simulink model "simulation_ref"  (R2026a)
settings: Solver=ode45  StopTime=stop_time  MaxStep=0.05
values from neighbouring files (symbols this model uses):
  throttle_trim = T_trim/T_max    [main.m]
undefined symbols (not defined in the file or in its folder): gravity_earth
settings Model: Creator=darpansingh  LastModifiedBy=lilos

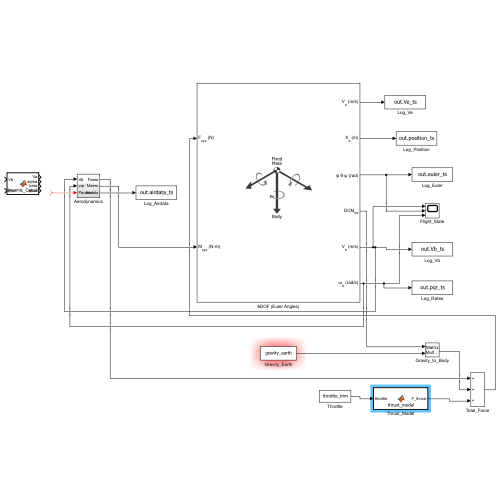
[thumbnail: Simulink's stored preview of the top-level diagram]
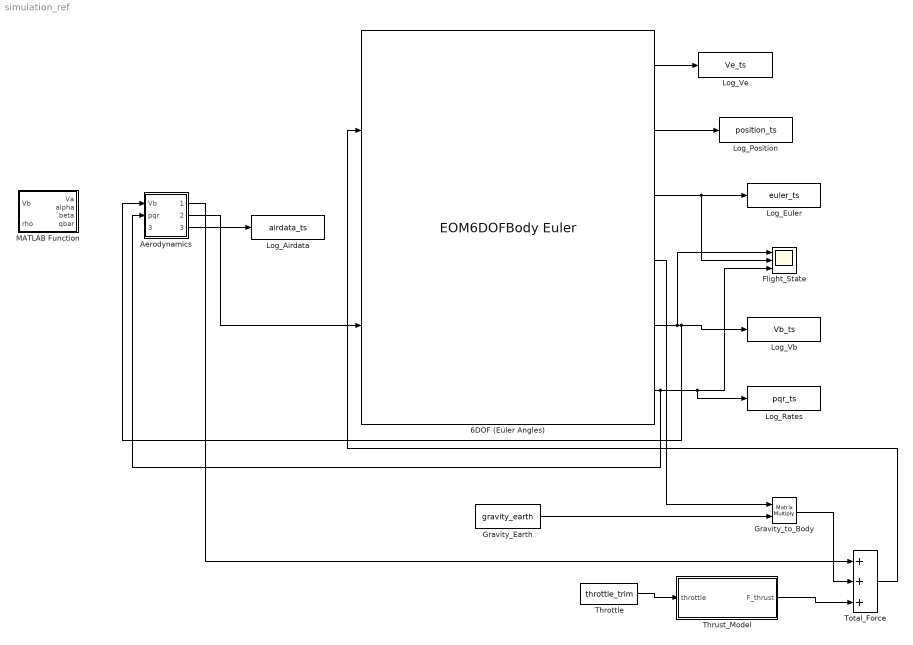
== system simulation_ref ==
  6DOF (Euler Angles) : EOM6DOFBodyEuler  xme_0=pos0  Vm_0=vel0  eul_0=euler0  pm_0=omega0  mass_0=mass  inertia=inertia
  Aerodynamics : Subsystem
  Flight_State : Scope  NumInputPorts=3
      settings: ActiveDisplayYMinimum=-1  ActiveDisplayYMaximum=1
  Gravity_Earth : Constant  Value=gravity_earth
  Gravity_to_Body : Product  Inputs=**  Multiplication=Matrix(*)
  Log_Airdata : ToWorkspace  VariableName=airdata_ts  SaveFormat=Timeseries  SampleTime=-1
  Log_Euler : ToWorkspace  VariableName=euler_ts  SaveFormat=Timeseries  SampleTime=-1
  Log_Position : ToWorkspace  VariableName=position_ts  SaveFormat=Timeseries  SampleTime=-1
  Log_Rates : ToWorkspace  VariableName=pqr_ts  SaveFormat=Timeseries  SampleTime=-1
  Log_Vb : ToWorkspace  VariableName=Vb_ts  SaveFormat=Timeseries  SampleTime=-1
  Log_Ve : ToWorkspace  VariableName=Ve_ts  SaveFormat=Timeseries  SampleTime=-1
  MATLAB Function : MATLAB Function  TreatAsAtomicUnit=on
  Throttle : Constant  Value=throttle_trim
  Thrust_Model : MATLAB Function  TreatAsAtomicUnit=on
  Total_Force : Sum  Inputs=+++
  wires:
  Aerodynamics/3(Airdata) -> Log_Airdata/1
  Aerodynamics/2(Maero) -> 6DOF (Euler Angles)/2
  Aerodynamics/1(Faero) -> Total_Force/1
  ? -> Aerodynamics/3(Params)
  6DOF (Euler Angles)/4 -> Gravity_to_Body/1
  Gravity_Earth/1 -> Gravity_to_Body/2
  Gravity_to_Body/1 -> Total_Force/2
  Total_Force/1 -> 6DOF (Euler Angles)/1
  6DOF (Euler Angles)/5 -> Log_Vb/1, Aerodynamics/1(Vb), Flight_State/1
  6DOF (Euler Angles)/3 -> Flight_State/2, Log_Euler/1
  6DOF (Euler Angles)/6 -> Flight_State/3, Log_Rates/1, Aerodynamics/2(pqr)
  6DOF (Euler Angles)/2 -> Log_Position/1
  6DOF (Euler Angles)/1 -> Log_Ve/1
  Throttle/1 -> Thrust_Model/1(throttle)
  Thrust_Model/1(F_thrust) -> Total_Force/3

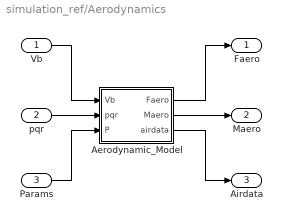
== system simulation_ref/Aerodynamics ==
  Vb : Inport
  pqr : Inport  Port=2
  Params : Inport  Port=3
  Aerodynamic_Model : MATLAB Function  TreatAsAtomicUnit=on
  Faero : Outport
  Maero : Outport  Port=2
  Airdata : Outport  Port=3
  wires:
  Aerodynamic_Model/3(airdata) -> Airdata/1
  Aerodynamic_Model/2(Maero) -> Maero/1
  Params/1 -> Aerodynamic_Model/3(P)
  pqr/1 -> Aerodynamic_Model/2(pqr)
  Vb/1 -> Aerodynamic_Model/1(Vb)
  Aerodynamic_Model/1(Faero) -> Faero/1

== matlab function simulation_ref/MATLAB Function ==
  data: Vb input; Va output; rho input; alpha output; beta output; qbar output

function [Va, alpha, beta, qbar] = Aerodynamic_Calculations(Vb, rho)

% Body-axis velocities
u = Vb(1);
v = Vb(2);
w = Vb(3);

% Airspeed (assuming no wind)
Va = sqrt(u^2 + v^2 + w^2);

% Angle of attack
alpha = atan2(w, u);

% Sideslip angle
beta = asin(max(-1, min(1, v/max(Va,1e-6))));

% Dynamic pressure
qbar = 0.5*rho*Va^2;

end

== matlab function simulation_ref/Aerodynamics/Aerodynamic_Model ==
  data: Vb input; Faero output; pqr input; P input; Maero output; airdata output
function [Faero, Maero, airdata] = aerodynamic_model(Vb, pqr, P)
%#codegen
u = Vb(1); v = Vb(2); w = Vb(3);
p = pqr(1); q = pqr(2); r = pqr(3);
rho = P(1); S = P(2); b = P(3); cbar = P(4); V0 = P(5);
CL0 = P(6); CL_V = P(7); CL_alpha = P(8); CL_q = P(9);
CD0 = P(10); k_drag = P(11); CD_V = P(12); CD_alpha = P(13);
Cm0 = P(14); Cm_V = P(15); Cm_alpha = P(16); Cm_q = P(17);
CY_beta = P(18); CY_p = P(19); CY_r = P(20);
Cl_beta = P(21); Cl_p = P(22); Cl_r = P(23);
Cn_beta = P(24); Cn_p = P(25); Cn_r = P(26);
Va = max(sqrt(u*u + v*v + w*w), 1.0);
alpha = atan2(w,u);
beta = asin(min(max(v/Va,-1.0),1.0));
dV = (Va - V0)/V0;
p_hat = p*b/(2*Va); q_hat = q*cbar/(2*Va); r_hat = r*b/(2*Va);
CL = CL0 + CL_V*dV + CL_alpha*alpha + CL_q*q_hat;
CD = CD0 + k_drag*CL*CL + CD_V*dV + CD_alpha*alpha;
Cm = Cm0 + Cm_V*dV + Cm_alpha*alpha + Cm_q*q_hat;
CY = CY_beta*beta + CY_p*p_hat + CY_r*r_hat;
Cl = Cl_beta*beta + Cl_p*p_hat + Cl_r*r_hat;
Cn = Cn_beta*beta + Cn_p*p_hat + Cn_r*r_hat;
qbar = 0.5*rho*Va*Va;
Lift = qbar*S*CL; Drag = qbar*S*CD; Side = qbar*S*CY;
ca = cos(alpha); sa = sin(alpha); cb = cos(beta); sb = sin(beta);
Xa = -Drag*ca*cb - Side*ca*sb + Lift*sa;
Ya = -Drag*sb + Side*cb;
Za = -Drag*sa*cb - Side*sa*sb - Lift*ca;
Faero = [Xa; Ya; Za];
Maero = [qbar*S*b*Cl; qbar*S*cbar*Cm; qbar*S*b*Cn];
airdata = [Va; alpha; beta; qbar; CL; CD];
end

== matlab function simulation_ref/Thrust_Model ==
  data: throttle input; F_thrust output size=3; T_max parameter
function F_thrust = thrust_model(throttle, T_max)
%#codegen
% Placeholder propulsion model: 4x P&W JT9D-3, LINEAR throttle law.
%   throttle : 0..1 command from the Throttle block (0 = idle, 1 = max)
%   T_max    : total max thrust at the trim condition [N] (parameter, set in main.m)
%   F_thrust : body-axis thrust force [N], along +x_b through the CG
% Replace the linear law with the JT9D throttle curve later.

th = min(max(throttle, 0), 1);   % clip to the physical lever range
F_thrust = [th*T_max; 0; 0];
end
